simulink model "H11_RC"  (R2026a)
settings: Solver=VariableStepAuto  StopTime=70e-3  MaxStep=R*C/25
InitFcn:
  | % Modellparaméterek
  | R = 100;
  | C = 10e-6;    % 10 uF
  | 
  | % Kezdeti érték
  | u_C0 = 5;
libraries: MK_H x4, simulink x1
settings Model: Creator=Szalay  LastModifiedBy=Szalay

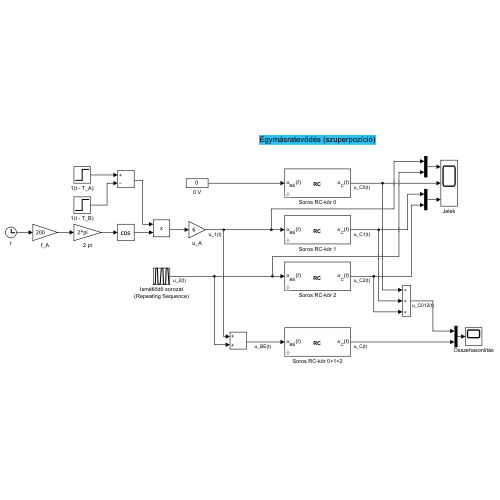
[thumbnail: Simulink's stored preview of the top-level diagram]
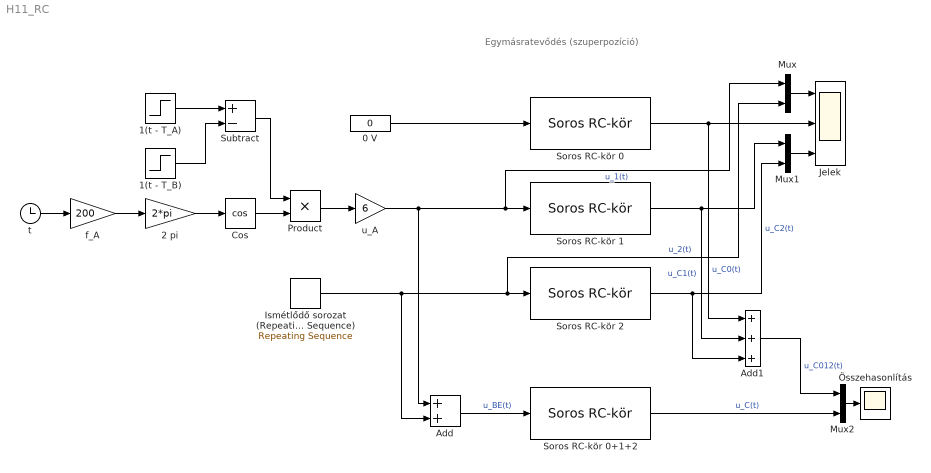
== system H11_RC ==
  note: Egymásratevődés (szuperpozíció)
  0 V : Constant  Value=0
  1(t - T_A) : Step  Time=10e-3  SampleTime=0
  1(t - T_B) : Step  Time=40e-3  SampleTime=0
  2 pi : Gain  Gain=2*pi
  Add : Sum
  Add1 : Sum  Inputs=+++
  Cos : Trigonometry  Operator=cos
  Ismétlődő sorozat (Repeating Sequence) : simulink/Sources/Repeating Sequence  rep_seq_t=[0, 20, 30, 50, 60, 70]*1e-3  rep_seq_y=[0, 0, 8, 8, 0, 0]
  Jelek : Scope  NumInputPorts=3
      settings: ActiveDisplayString=3  ActiveDisplayYMinimum=-5.3101009449866465  ActiveDisplayYMaximum=9.4887505408870219
  Mux : Mux  Inputs=2
  Mux1 : Mux  Inputs=2
  Mux2 : Mux  Inputs=2
  Product : Product
  Soros RC-kör 0 : MK_H/Soros RC-kör  R=R  C=C  u_C0=u_C0
  Soros RC-kör 0+1+2 : MK_H/Soros RC-kör  R=R  C=C  u_C0=u_C0
  Soros RC-kör 1 : MK_H/Soros RC-kör  R=R  C=C  u_C0=0
  Soros RC-kör 2 : MK_H/Soros RC-kör  R=R  C=C  u_C0=0
  Subtract : Sum  Inputs=+-
  f_A : Gain  Gain=200
  t : Clock
  u_A : Gain  Gain=6
  Összehasonlítás : Scope
      settings: ActiveDisplayYMinimum=-5.77565334179253  ActiveDisplayYMaximum=13.678814642199896
  wires:
  0 V/1 -> Soros RC-kör 0/1
  u_A/1 -> Add/1, Mux/1, Soros RC-kör 1/1  "u_1(t)"
  Product/1 -> u_A/1
  1(t - T_A)/1 -> Subtract/1
  1(t - T_B)/1 -> Subtract/2
  Subtract/1 -> Product/1
  Cos/1 -> Product/2
  2 pi/1 -> Cos/1
  f_A/1 -> 2 pi/1
  t/1 -> f_A/1
  Soros RC-kör 0/1 -> Jelek/2, Add1/1  "u_C0(t)"
  Soros RC-kör 1/1 -> Add1/2, Mux1/1  "u_C1(t)"
  Ismétlődő sorozat (Repeating Sequence)/1 -> Add/2, Mux/2, Soros RC-kör 2/1  "u_2(t)"
  Mux/1 -> Jelek/1
  Mux1/1 -> Jelek/3
  Soros RC-kör 2/1 -> Add1/3, Mux1/2  "u_C2(t)"
  Add/1 -> Soros RC-kör 0+1+2/1  "u_BE(t)"
  Mux2/1 -> Összehasonlítás/1
  Soros RC-kör 0+1+2/1 -> Mux2/2  "u_C(t)"
  Add1/1 -> Mux2/1  "u_C012(t)"
